simulink model "Partie4_Hamming"  (R2026b)
settings: Solver=FixedStepDiscrete  StopTime=Tstop_Q10
undefined symbols (not defined in the file): A_code, graine, graine_bruit, p1, Tb, variance_bruit_code
libraries: simulink x1
settings Model: Creator=WORLD COMPUTERS  LastModifiedBy=WORLD COMPUTERS

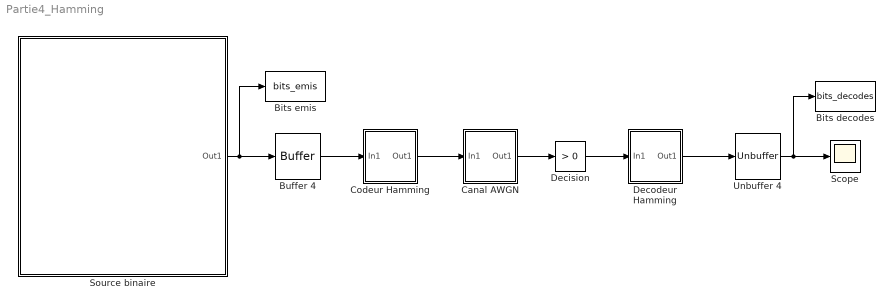
== system Partie4_Hamming ==
  Bits decodes : ToWorkspace  VariableName=bits_decodes  SampleTime=-1
  Bits emis : ToWorkspace  VariableName=bits_emis  SampleTime=-1
  Buffer 4 : Buffer  N=4
  Canal AWGN : Subsystem
  Codeur Hamming : Subsystem
  Decision : simulink/Logic and Bit Operations/Compare To Constant  relop=>  const=0  OutDataTypeStr=boolean
  Decodeur Hamming : Subsystem
  Scope : Scope
  Source binaire : Subsystem
  Unbuffer 4 : Unbuffer
  wires:
  Canal AWGN/1(Out1) -> Decision/1
  Buffer 4/1 -> Codeur Hamming/1(In1)
  Source binaire/1(Out1) -> Buffer 4/1, Bits emis/1
  Unbuffer 4/1 -> Bits decodes/1, Scope/1
  Decision/1 -> Decodeur Hamming/1(In1)
  Codeur Hamming/1(Out1) -> Canal AWGN/1(In1)
  Decodeur Hamming/1(Out1) -> Unbuffer 4/1

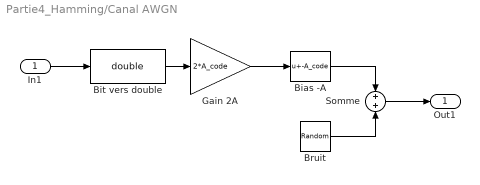
== system Partie4_Hamming/Canal AWGN ==
  In1 : Inport
  Bias -A : Bias  Bias=-A_code  SaturateOnIntegerOverflow=off
  Bit vers double : DataTypeConversion  OutDataTypeStr=double  SaturateOnIntegerOverflow=off  RndMeth=Floor
  Bruit : RandomNumber  Variance=variance_bruit_code*ones(7,1)  Seed=graine_bruit+(1:7)'  SampleTime=4*Tb
  Gain 2A : Gain  Gain=2*A_code
  Somme : Sum
  Out1 : Outport
  wires:
  In1/1 -> Bit vers double/1
  Bias -A/1 -> Somme/1
  Gain 2A/1 -> Bias -A/1
  Bit vers double/1 -> Gain 2A/1
  Somme/1 -> Out1/1
  Bruit/1 -> Somme/2

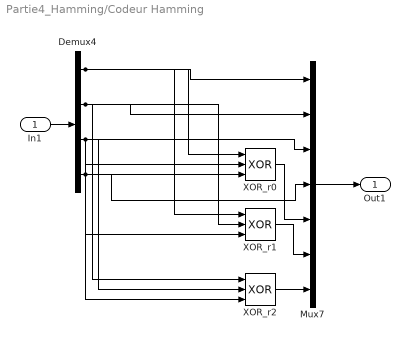
== system Partie4_Hamming/Codeur Hamming ==
  In1 : Inport
  Demux4 : Demux
  Mux7 : Mux  Inputs=7
  XOR_r0 : Logic  Operator=XOR  Inputs=3  AllPortsSameDT=off  OutDataTypeStr=boolean
  XOR_r1 : Logic  Operator=XOR  Inputs=3  AllPortsSameDT=off  OutDataTypeStr=boolean
  XOR_r2 : Logic  Operator=XOR  Inputs=3  AllPortsSameDT=off  OutDataTypeStr=boolean
  Out1 : Outport
  wires:
  In1/1 -> Demux4/1
  Demux4/4 -> Mux7/4, XOR_r0/3, XOR_r2/3
  Demux4/3 -> Mux7/3, XOR_r0/2, XOR_r1/3, XOR_r2/2
  Demux4/2 -> Mux7/2, XOR_r1/2, XOR_r2/1
  Demux4/1 -> Mux7/1, XOR_r0/1, XOR_r1/1
  XOR_r0/1 -> Mux7/5
  XOR_r2/1 -> Mux7/7
  XOR_r1/1 -> Mux7/6
  Mux7/1 -> Out1/1

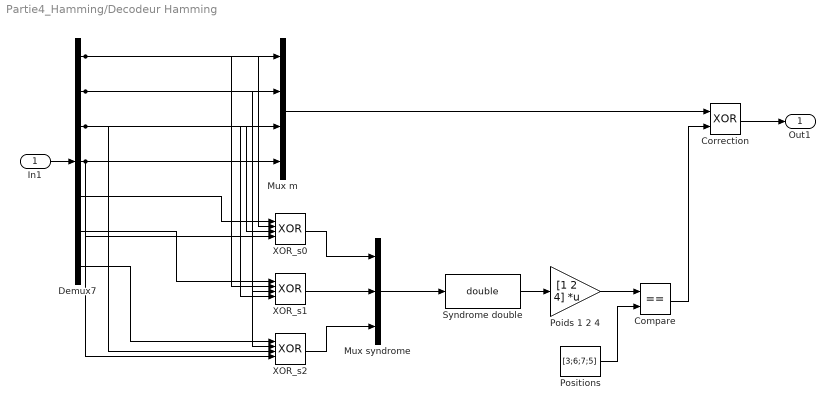
== system Partie4_Hamming/Decodeur Hamming ==
  In1 : Inport
  Compare : RelationalOperator  Operator===  OutDataTypeStr=boolean  RndMeth=Simplest  InputSameDT=off
  Correction : Logic  Operator=XOR  AllPortsSameDT=off  OutDataTypeStr=boolean
  Demux7 : Demux  Outputs=7
  Mux m : Mux
  Mux syndrome : Mux  Inputs=3
  Poids 1 2 4 : Gain  Gain=[1 2 4]  Multiplication=Matrix(K*u)
  Positions : Constant  Value=[3;6;7;5]
  Syndrome double : DataTypeConversion  OutDataTypeStr=double  SaturateOnIntegerOverflow=off  RndMeth=Floor
  XOR_s0 : Logic  Operator=XOR  Inputs=4  AllPortsSameDT=off  OutDataTypeStr=boolean
  XOR_s1 : Logic  Operator=XOR  Inputs=4  AllPortsSameDT=off  OutDataTypeStr=boolean
  XOR_s2 : Logic  Operator=XOR  Inputs=4  AllPortsSameDT=off  OutDataTypeStr=boolean
  Out1 : Outport
  wires:
  In1/1 -> Demux7/1
  XOR_s2/1 -> Mux syndrome/3
  Demux7/7 -> XOR_s2/1
  Demux7/6 -> XOR_s1/1
  Mux syndrome/1 -> Syndrome double/1
  Demux7/5 -> XOR_s0/1
  Demux7/4 -> XOR_s0/4, XOR_s2/4, Mux m/4
  XOR_s0/1 -> Mux syndrome/1
  Demux7/3 -> XOR_s0/3, XOR_s1/4, XOR_s2/3, Mux m/3
  Demux7/2 -> XOR_s1/3, XOR_s2/2, Mux m/2
  XOR_s1/1 -> Mux syndrome/2
  Demux7/1 -> XOR_s0/2, XOR_s1/2, Mux m/1
  Poids 1 2 4/1 -> Compare/1
  Mux m/1 -> Correction/1
  Syndrome double/1 -> Poids 1 2 4/1
  Compare/1 -> Correction/2
  Positions/1 -> Compare/2
  Correction/1 -> Out1/1

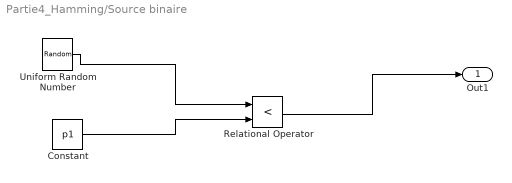
== system Partie4_Hamming/Source binaire ==
  Constant : Constant  Value=p1
  Relational Operator : RelationalOperator  Operator=<  OutDataTypeStr=boolean  RndMeth=Simplest  InputSameDT=off
  Uniform Random Number : UniformRandomNumber  Minimum=0  Seed=graine  SampleTime=Tb
  Out1 : Outport
  wires:
  Relational Operator/1 -> Out1/1
  Constant/1 -> Relational Operator/2
  Uniform Random Number/1 -> Relational Operator/1
